simulink library "lib_SecCtrl_MatricesDelay"  (R2026a)
settings: Solver=VariableStepAuto
undefined symbols (not defined in the file): A_f_sc, A_P_sc, A_Q_sc, A_v_sc, buses_lf, delayM
settings Model: Creator=atomas  LastModifiedBy=atomas

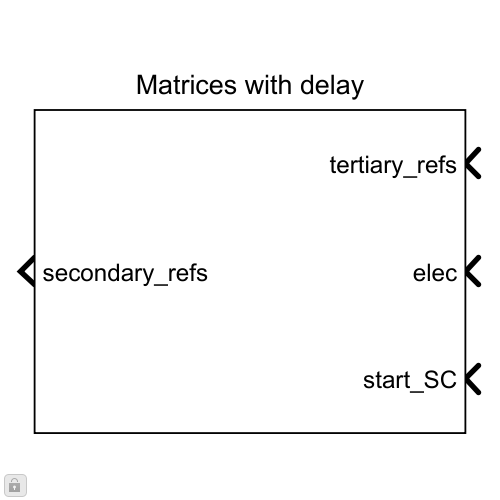
[thumbnail: Simulink's stored preview of the top-level diagram]
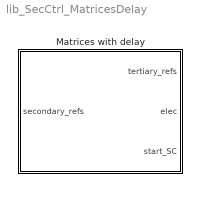
== system lib_SecCtrl_MatricesDelay ==
  Matrices with delay : Subsystem  VariantControl=Matrices with delay

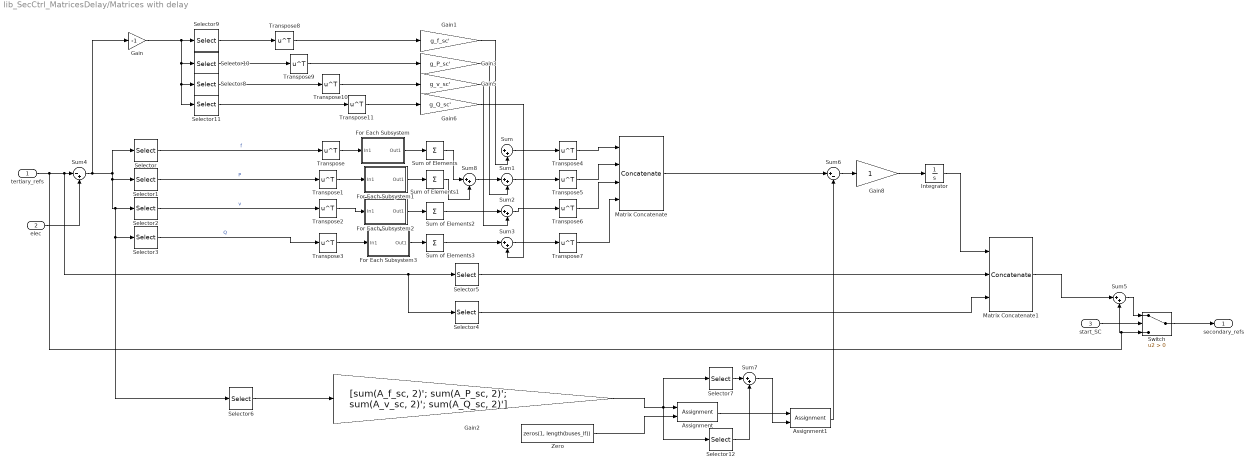
== system lib_SecCtrl_MatricesDelay/Matrices with delay ==
  tertiary_refs : Inport
  elec : Inport  Port=2
  start_SC : Inport  Port=3
  Assignment : Assignment  NumberOfDimensions=2  DiagnosticForDimensions=Warning  IndexOptions=Index vector (dialog),Assign all  Indices=1,1  OutputSizes=1,1
  Assignment1 : Assignment  NumberOfDimensions=2  DiagnosticForDimensions=Warning  IndexOptions=Index vector (dialog),Assign all  Indices=2,1  OutputSizes=1,1
  For Each Subsystem : Subsystem  TreatAsAtomicUnit=on  mask{delayM=delayM, A_f_sc=A_f_sc}
  For Each Subsystem1 : Subsystem  TreatAsAtomicUnit=on  mask{delayM=delayM, A_P_sc=A_P_sc}
  For Each Subsystem2 : Subsystem  TreatAsAtomicUnit=on  mask{delayM=delayM, A_v_sc=A_v_sc}
  For Each Subsystem3 : Subsystem  TreatAsAtomicUnit=on  mask{delayM=delayM, A_Q_sc=A_Q_sc}
  Gain : Gain  Gain=-1
  Gain1 : Gain  Gain=g_f_sc'
  Gain2 : Gain  Gain=[sum(A_f_sc, 2)'; sum(A_P_sc, 2)'; sum(A_v_sc, 2)'; sum(A_Q_sc, 2)']
  Gain3 : Gain  Gain=g_P_sc'
  Gain5 : Gain  Gain=g_v_sc'
  Gain6 : Gain  Gain=g_Q_sc'
  Gain8 : Gain
  Integrator : Integrator
  Matrix Concatenate : Concatenate  NumInputs=4  Mode=Multidimensional array
  Matrix Concatenate1 : Concatenate  NumInputs=3  Mode=Multidimensional array
  Selector : Selector  NumberOfDimensions=2  InputPortWidth=3  IndexOptions=Index vector (dialog),Select all  Indices=1,1  OutputSizes=1,1
  Selector1 : Selector  NumberOfDimensions=2  InputPortWidth=3  IndexOptions=Index vector (dialog),Select all  Indices=2,1  OutputSizes=1,1
  Selector10 : Selector  NumberOfDimensions=2  InputPortWidth=3  IndexOptions=Index vector (dialog),Select all  Indices=2,1  OutputSizes=1,1
  Selector11 : Selector  NumberOfDimensions=2  InputPortWidth=3  IndexOptions=Index vector (dialog),Select all  Indices=4,1  OutputSizes=1,1
  Selector12 : Selector  NumberOfDimensions=2  InputPortWidth=3  IndexOptions=Index vector (dialog),Select all  Indices=2,1  OutputSizes=1,1
  Selector2 : Selector  NumberOfDimensions=2  InputPortWidth=3  IndexOptions=Index vector (dialog),Select all  Indices=3,1  OutputSizes=1,1
  Selector3 : Selector  NumberOfDimensions=2  InputPortWidth=3  IndexOptions=Index vector (dialog),Select all  Indices=4,1  OutputSizes=1,1
  Selector4 : Selector  NumberOfDimensions=2  InputPortWidth=3  IndexOptions=Index vector (dialog),Select all  Indices=6,1  OutputSizes=1,1
  Selector5 : Selector  NumberOfDimensions=2  InputPortWidth=3  IndexOptions=Index vector (dialog),Select all  Indices=5,1  OutputSizes=1,1
  Selector6 : Selector  NumberOfDimensions=2  InputPortWidth=3  IndexOptions=Index vector (dialog),Select all  Indices=1:4,1  OutputSizes=1,1
  Selector7 : Selector  NumberOfDimensions=2  InputPortWidth=3  IndexOptions=Index vector (dialog),Select all  Indices=1,1  OutputSizes=1,1
  Selector8 : Selector  NumberOfDimensions=2  InputPortWidth=3  IndexOptions=Index vector (dialog),Select all  Indices=3,1  OutputSizes=1,1
  Selector9 : Selector  NumberOfDimensions=2  InputPortWidth=3  IndexOptions=Index vector (dialog),Select all  Indices=1,1  OutputSizes=1,1
  Sum{,1..3,5,7..8} (7 alike) : Sum  Inputs=|++
  Sum of Elements{,1..3} (4 alike) : Sum  Inputs=+  CollapseMode=Specified dimension  CollapseDim=2
  Sum4 : Sum  Inputs=|-+
  Sum6 : Sum  Inputs=|+-
  Switch : Switch  Criteria=u2 > Threshold  SaturateOnIntegerOverflow=off  InputSameDT=off
  Transpose{,1..11} (12 alike) : Math  Operator=transpose
  Zero : Constant  Value=zeros(1, length(buses_lf))  VectorParams1D=off  OutDataTypeStr=Inherit: Inherit via back propagation
  secondary_refs : Outport
  wires:
  Sum of Elements1/1 -> Sum8/2
  Sum8/1 -> Sum1/1
  Sum of Elements/1 -> Sum8/1
  Assignment1/1 -> Sum6/2
  Sum7/1 -> Assignment1/2
  Selector12/1 -> Sum7/2
  Selector7/1 -> Sum7/1
  Assignment/1 -> Assignment1/1
  Zero/1 -> Assignment/2
  Gain2/1 -> Assignment/1, Selector12/1, Selector7/1
  Selector5/1 -> Matrix Concatenate1/2
  Gain8/1 -> Integrator/1
  Integrator/1 -> Matrix Concatenate1/1
  Gain/1 -> Selector9/1, Selector10/1, Selector8/1, Selector11/1
  Transpose11/1 -> Gain6/1
  Transpose10/1 -> Gain5/1
  Transpose9/1 -> Gain3/1
  Transpose8/1 -> Gain1/1
  start_SC/1 -> Switch/2
  Selector6/1 -> Gain2/1
  Matrix Concatenate/1 -> Sum6/1
  Sum6/1 -> Gain8/1
  Selector9/1 -> Transpose8/1
  Sum4/1 -> Selector/1, Selector1/1, Selector3/1, Selector6/1, Selector2/1, Gain/1
  Selector11/1 -> Transpose11/1
  Selector8/1 -> Transpose10/1
  Selector10/1 -> Transpose9/1
  Sum5/1 -> Switch/1
  Matrix Concatenate1/1 -> Sum5/1
  elec/1 -> Sum4/2
  tertiary_refs/1 -> Sum4/1, Selector5/1, Selector4/1, Switch/3, Sum5/2
  Transpose5/1 -> Matrix Concatenate/2
  Switch/1 -> secondary_refs/1
  For Each Subsystem3/1(Out1) -> Sum of Elements3/1
  For Each Subsystem2/1(Out1) -> Sum of Elements2/1
  For Each Subsystem1/1(Out1) -> Sum of Elements1/1
  For Each Subsystem/1(Out1) -> Sum of Elements/1
  Transpose7/1 -> Matrix Concatenate/4
  Transpose6/1 -> Matrix Concatenate/3
  Transpose4/1 -> Matrix Concatenate/1
  Transpose3/1 -> For Each Subsystem3/1(In1)
  Transpose2/1 -> For Each Subsystem2/1(In1)
  Transpose1/1 -> For Each Subsystem1/1(In1)
  Transpose/1 -> For Each Subsystem/1(In1)
  Sum of Elements3/1 -> Sum3/1
  Sum3/1 -> Transpose7/1
  Sum2/1 -> Transpose6/1
  Gain6/1 -> Sum3/2
  Gain5/1 -> Sum2/2
  Sum of Elements2/1 -> Sum2/1
  Sum1/1 -> Transpose5/1
  Gain3/1 -> Sum1/2
  Gain1/1 -> Sum/2
  Sum/1 -> Transpose4/1
  Selector4/1 -> Matrix Concatenate1/3
  Selector2/1 -> Transpose2/1  "v"
  Selector1/1 -> Transpose1/1  "P"
  Selector/1 -> Transpose/1  "f"
  Selector3/1 -> Transpose3/1  "Q"

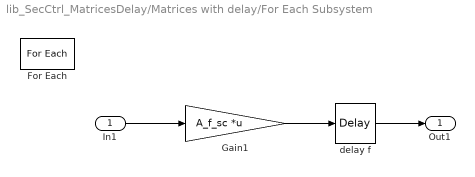
== system lib_SecCtrl_MatricesDelay/Matrices with delay/For Each Subsystem ==
  In1 : Inport  Partition=on  PartitionDimension=1  PartitionWidth=1  PartitionOffset=0
  For Each : ForEach  DisableCoverage=on  IterateSubsysMaskParameter=on,on  SubsysMaskParameterIterationDimension=2,2
  Gain1 : Gain  Gain=A_f_sc  Multiplication=Matrix(K*u)
  delay f : TransportDelay  DelayTime=delayM  PadeOrder=3
  Out1 : Outport  ConcatenationDimension=2
  wires:
  delay f/1 -> Out1/1
  In1/1 -> Gain1/1
  Gain1/1 -> delay f/1

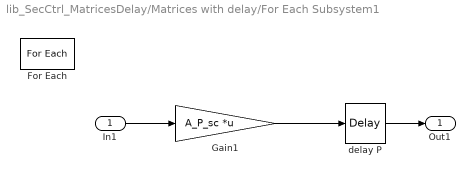
== system lib_SecCtrl_MatricesDelay/Matrices with delay/For Each Subsystem1 ==
  In1 : Inport  Partition=on  PartitionDimension=1  PartitionWidth=1  PartitionOffset=0
  For Each : ForEach  DisableCoverage=on  IterateSubsysMaskParameter=on,on  SubsysMaskParameterIterationDimension=2,2
  Gain1 : Gain  Gain=A_P_sc  Multiplication=Matrix(K*u)
  delay P : TransportDelay  DelayTime=delayM  PadeOrder=3
  Out1 : Outport  ConcatenationDimension=2
  wires:
  Gain1/1 -> delay P/1
  In1/1 -> Gain1/1
  delay P/1 -> Out1/1

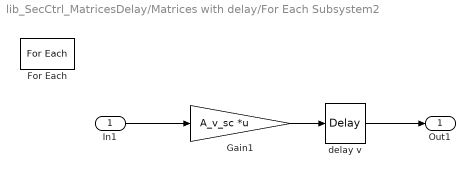
== system lib_SecCtrl_MatricesDelay/Matrices with delay/For Each Subsystem2 ==
  In1 : Inport  Partition=on  PartitionDimension=1  PartitionWidth=1  PartitionOffset=0
  For Each : ForEach  DisableCoverage=on  IterateSubsysMaskParameter=on,on  SubsysMaskParameterIterationDimension=2,2
  Gain1 : Gain  Gain=A_v_sc  Multiplication=Matrix(K*u)
  delay v : TransportDelay  DelayTime=delayM  PadeOrder=3
  Out1 : Outport  ConcatenationDimension=2
  wires:
  Gain1/1 -> delay v/1
  delay v/1 -> Out1/1
  In1/1 -> Gain1/1

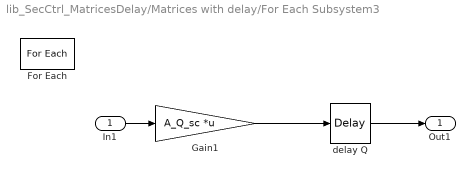
== system lib_SecCtrl_MatricesDelay/Matrices with delay/For Each Subsystem3 ==
  In1 : Inport  Partition=on  PartitionDimension=1  PartitionWidth=1  PartitionOffset=0
  For Each : ForEach  DisableCoverage=on  IterateSubsysMaskParameter=on,on  SubsysMaskParameterIterationDimension=2,2
  Gain1 : Gain  Gain=A_Q_sc  Multiplication=Matrix(K*u)
  delay Q : TransportDelay  DelayTime=delayM  PadeOrder=3
  Out1 : Outport  ConcatenationDimension=2
  wires:
  delay Q/1 -> Out1/1
  In1/1 -> Gain1/1
  Gain1/1 -> delay Q/1
